simulink model "BMS_controller"  (R2024a)
settings: Solver=ode1  StartTime=0.0  StopTime=1800  FixedStep=0.01  RelTol=1e-3  EnableMultiTasking=on
InitFcn:
  | init_bms;
settings Model: SILPILSystemUnderTest=refmodels  Creator=Lenovo  LastModifiedBy=Lenovo
settings OptimizationCC: EnhancedBackFolding=on  PassReuseOutputArgsAs=Individual arguments  ZeroExternalMemoryAtStartup=off  ZeroInternalMemoryAtStartup=off  MaxStackSize=64  OptimizeBlockOrder=speed  DifferentSizesBufferReuse=on  OptimizationCustomize=off  EfficientTunableParamExpr=on
settings DebuggingCC: ParameterTunabilityLossMsg=error
settings HardwareCC: ProdBitPerPointer=32  ProdBitPerSizeT=32  ProdBitPerPtrDiffT=32  ProdLargestAtomicInteger=Long  ProdLargestAtomicFloat=Double  ProdWordSize=32  ProdLongLongMode=on  ProdHWDeviceType=ARM Compatible->ARM Cortex-M
settings ModelReferenceCC: UpdateModelReferenceTargets=Force
settings SFSimCC: MATLABDynamicMemAlloc=off
settings RTWCC: Description=Embedded Coder  SystemTargetFile=ert.tlc  HardwareBoard=STM32L4xx Based  TemplateMakefile=ert_default_tmf  Toolchain=GNU Tools for ARM Embedded Processors  CodeExecutionProfiling=on
settings CodeAppCC: ForceParamTrailComments=on  IgnoreCustomStorageClasses=off  OperatorAnnotations=on  SimulinkDataObjDesc=on  SFDataObjDesc=on  InsertBlockDesc=on
settings ERTTargetCC: TargetLangStandard=C99 (ISO)  CodeReplacementLibrary=ARM Cortex-M  ExtModeTransport=3  ExtModeStaticAlloc=on  ExtModeStaticAllocSize=2048  ExtModeMexFile=ext_xcp  ExtModeIntrfLevel=Level2 - Open
settings ConfigComp: CovEnable=on  RecordCoverage=on  CovSaveName=covdata_SIL  CovMetricSettings=dcm  CovModelRefEnable=all

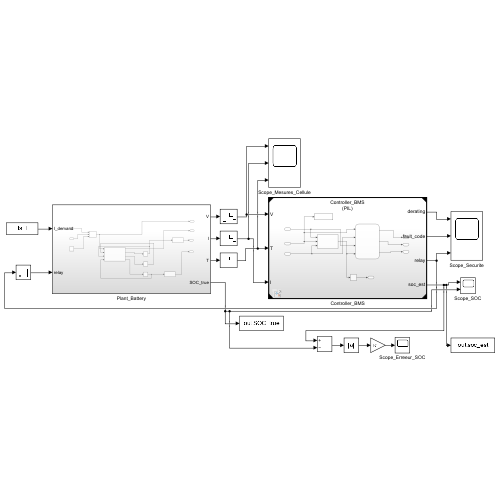
[thumbnail: Simulink's stored preview of the top-level diagram]
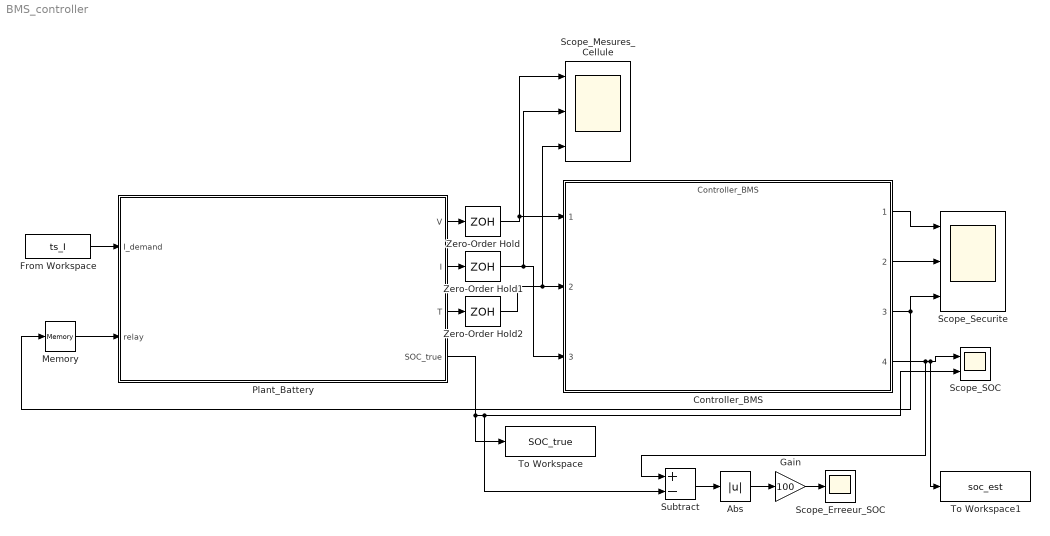
== system BMS_controller ==
  Abs : Abs  SaturateOnIntegerOverflow=off
  Controller_BMS : ModelReference  ModelNameDialog=Controller_BMS  SimulationMode=Processor-in-the-loop (PIL)  ModelReferenceVersion=1.63
  From Workspace : FromWorkspace  VariableName=ts_I
  Gain : Gain  Gain=100
  Memory : Memory  InitialCondition=single(1)
  Plant_Battery : Subsystem
  Scope_Erreeur_SOC : Scope
  Scope_Mesures_Cellule : Scope  NumInputPorts=3
  Scope_SOC : Scope  NumInputPorts=2
  Scope_Securite : Scope  NumInputPorts=3
  Subtract : Sum  Inputs=+-
  To Workspace : ToWorkspace  VariableName=SOC_true  SampleTime=-1
  To Workspace1 : ToWorkspace  VariableName=soc_est  SampleTime=-1
  Zero-Order Hold : ZeroOrderHold  SampleTime=0.01
  Zero-Order Hold1 : ZeroOrderHold  SampleTime=0.01
  Zero-Order Hold2 : ZeroOrderHold  SampleTime=0.01
  wires:
  Controller_BMS/1 -> Scope_Securite/1
  Controller_BMS/2 -> Scope_Securite/2
  Controller_BMS/3 -> Memory/1, Scope_Securite/3
  From Workspace/1 -> Plant_Battery/1(I_demand)
  Plant_Battery/4(SOC_true) -> To Workspace/1, Scope_SOC/2, Subtract/2
  Subtract/1 -> Abs/1
  Controller_BMS/4 -> To Workspace1/1, Scope_SOC/1, Subtract/1
  Abs/1 -> Gain/1
  Gain/1 -> Scope_Erreeur_SOC/1
  Memory/1 -> Plant_Battery/2(relay)
  Plant_Battery/1(V) -> Zero-Order Hold/1
  Zero-Order Hold/1 -> Scope_Mesures_Cellule/1, Controller_BMS/1
  Plant_Battery/2(I) -> Zero-Order Hold1/1
  Plant_Battery/3(T) -> Zero-Order Hold2/1
  Zero-Order Hold1/1 -> Scope_Mesures_Cellule/2, Controller_BMS/3
  Zero-Order Hold2/1 -> Scope_Mesures_Cellule/3, Controller_BMS/2

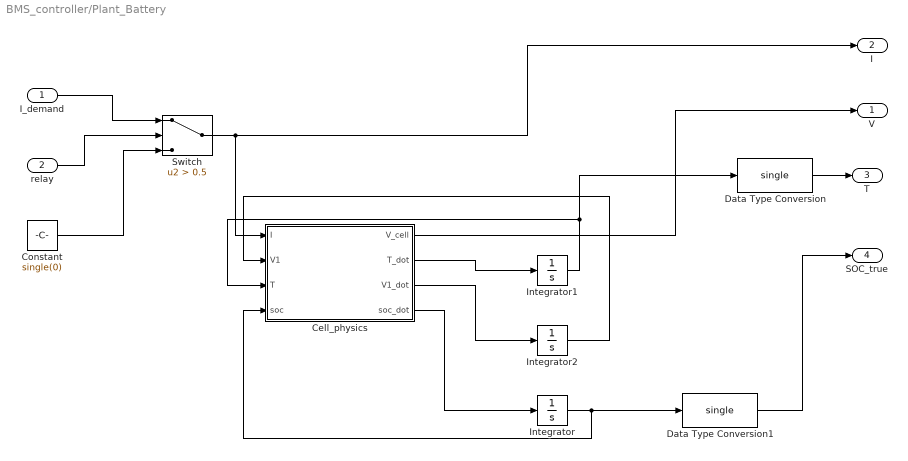
== system BMS_controller/Plant_Battery ==
  I_demand : Inport
  relay : Inport  Port=2
  Cell_physics : MATLAB Function  TreatAsAtomicUnit=on
  Constant : Constant  Value=single(0)
  Data Type Conversion : DataTypeConversion  OutDataTypeStr=single  SaturateOnIntegerOverflow=off  RndMeth=Floor
  Data Type Conversion1 : DataTypeConversion  OutDataTypeStr=single  SaturateOnIntegerOverflow=off  RndMeth=Floor
  Integrator : Integrator  InitialCondition=0.95
  Integrator1 : Integrator  InitialCondition=25
  Integrator2 : Integrator
  Switch : Switch  Criteria=u2 > Threshold  Threshold=0.5  SaturateOnIntegerOverflow=off  InputSameDT=off
  V : Outport
  I : Outport  Port=2
  T : Outport  Port=3
  SOC_true : Outport  Port=4
  wires:
  I_demand/1 -> Switch/1
  relay/1 -> Switch/2
  Constant/1 -> Switch/3
  Switch/1 -> Cell_physics/1(I), I/1
  Cell_physics/2(T_dot) -> Integrator1/1
  Cell_physics/3(V1_dot) -> Integrator2/1
  Cell_physics/4(soc_dot) -> Integrator/1
  Integrator/1 -> Data Type Conversion1/1, Cell_physics/4(soc)
  Integrator2/1 -> Cell_physics/2(V1)
  Integrator1/1 -> Data Type Conversion/1, Cell_physics/3(T)
  Cell_physics/1(V_cell) -> V/1
  Data Type Conversion/1 -> T/1
  Data Type Conversion1/1 -> SOC_true/1

== matlab function BMS_controller/Plant_Battery/Cell_physics ==
  data: I input; V_cell output; V1 input; T input; soc input; T_dot output; V1_dot output; soc_dot output
function [V_cell, T_dot, V1_dot, soc_dot] = cell_physics(I, V1, T, soc)
%#codegen

% =========================================================================
% 1. PARAMETRES PHYSIQUES DE LA CELLULE (Identiques a CELLULE.m)
% =========================================================================
Cn    = 2.5 * 3600.0; % Capacite nominale en Coulombs (As) [2.5 Ah]
R0    = 0.025;        % Resistance serie ohmique (Ohm)
R1    = 0.015;        % Resistance de polarisation (Ohm)
C1    = 1500.0;       % Capacite de polarisation (Farad)
C_th  = 65.0;         % Capacite thermique (J/K)
hA    = 0.080;        % Coefficient de convection thermique (W/K)
T_amb = 25.0;         % Temperature ambiante (degC)

% =========================================================================
% 2. CONVERSION DES ENTREES EN DOUBLE (Pour la precision du solveur continu)
% =========================================================================
I_d   = double(I);
V1_d  = double(V1);
T_d   = double(T);
soc_d = double(soc);

% Saturation de securite du SOC entre 0 et 1
soc_clamped = min(max(soc_d, 0.0), 1.0);

% =========================================================================
% 3. TENSION A VIDE Voc PAR LOOK-UP TABLE (Remplacement du polynome)
% =========================================================================
soc_pts = [0.0,  0.10, 0.20, 0.30, 0.40, 0.50, 0.60, 0.70, 0.80, 0.90, 1.0];
ocv_pts = [3.00, 3.45, 3.62, 3.68, 3.74, 3.80, 3.87, 3.95, 4.05, 4.14, 4.20];

% Interpolation lineaire compatible Coder / Simulink
Voc = interp1(soc_pts, ocv_pts, soc_clamped, 'linear');

% =========================================================================
% 4. EQUATIONS D'ETAT CONTINUES (Derivees pour les integrateurs 1/s)
% =========================================================================
% Dynamique thermique : Echauffement par effet Joule - Pertes par convection
T_dot   = (R0 * (I_d^2) - hA * (T_d - T_amb)) / C_th;

% Dynamique du circuit RC (Tension de polarisation V1)
V1_dot  = (-1.0 / (R1 * C1)) * V1_d + (1.0 / C1) * I_d;

% Coulomb Counting pour le vrai SOC
soc_dot = -I_d / Cn;

% =========================================================================
% 5. TENSION DE SORTIE MESUREE AUX BORNES DE LA CELLULE
% =========================================================================
% V_cell = Voc - R0*I - V1
V_cell  = single(Voc - R0 * I_d - V1_d);

end
